simulink model "hex_simulation_standing"  (R2026a)
settings: Solver=VariableStepAuto  StopTime=9
model workspace: external: MATLAB File simscape_data.m (data not in the file)
undefined symbols (not defined in the file or in its folder): smiData, X, Y, Z
libraries: sm_lib x398, nesl_utility x23
(part 7 of 7)

== system hex_simulation_standing/Right Back/Complete_servo_assembly_3_RIGID/Servo_Horn_1_RIGID ==
  ReferenceFrame : sm_lib/Frames and Transforms/Reference Frame
  Solid : sm_lib/Body Elements/File Solid  ExtGeomFileName=servo-horn.step  UnitType=FromFile  ExtGeomFileUnits=m  StepReaderType=HEX  ExportConvexHullGeometry=off  InertiaType=Custom  BasedOnType=DensityFromFile  Density=1000  DensityUnits=kg/m^3  Mass=smiData.Solid(3).mass  MassUnits=kg  CenterOfMass=smiData.Solid(3).CoM  CenterOfMassUnits=mm  MomentsOfInertia=smiData.Solid(3).MoI  MomentsOfInertiaUnits=kg*mm^2  ProductsOfInertia=smiData.Solid(3).PoI  ProductsOfInertiaUnits=kg*mm^2  GraphicType=FromGeometry  MarkerShape=Sphere  MarkerSize=10  GraphicVisPropType=SimpleVisualProperties  GraphicDiffuseColor=smiData.Solid(3).color  GraphicOpacity=smiData.Solid(3).opacity  GraphicSpecularColor=[0.5 0.5 0.5 1.0]  GraphicAmbientColor=[0.15 0.15 0.15 1.0]  GraphicEmissiveColor=[0.0 0.0 0.0 1.0]  GraphicShininess=75  DoExposeReferenceFrame=on  SerializedFrames=<Frames/>
  F : PMIOPort  Side=Left
  connections:
  Solid/RConn1 -- ReferenceFrame/RConn1 -- F/RConn1

== system hex_simulation_standing/Right Front/Complete_servo_assembly_1_RIGID/Assem3Complete_servo_assembly_1_RIGID ==
  ReferenceFrame : sm_lib/Frames and Transforms/Reference Frame
  Transform : sm_lib/Frames and Transforms/Rigid Transform  RotationMethod=ArbitraryAxis  FollAlignAxisA=+X  BaseAlignAxisA=+Y  FollAlignAxisB=+Y  BaseAlignAxisB=+Z  RotationStandardAxis=+Z  RotationAngle=smiData.RigidTransform(74).angle  RotationAngleUnits=rad  RotationArbitraryAxis=smiData.RigidTransform(74).axis  RotationSequenceAxes=FollowerAxes  RotationSequence=XYX  RotationSequenceAngles=[0 0 0]  RotationSequenceAnglesUnits=deg  RotationMatrix=[1 0 0;0 1 0;0 0 1]  Quaternion=[1 0 0 0]  TranslationMethod=Cartesian  TranslationCartesianOffset=smiData.RigidTransform(74).translation  TranslationCartesianOffsetUnits=mm  TranslationStandardAxis=+Z  TranslationStandardOffset=0  TranslationStandardOffsetUnits=m  TranslationROffset=0  TranslationROffsetUnits=m  TranslationThetaOffset=0  TranslationThetaOffsetUnits=deg  TranslationZOffset=0  TranslationZOffsetUnits=m
  F : PMIOPort  Side=Right
  connections:
  ReferenceFrame/RConn1 -- Transform/RConn1
  Transform/LConn1 -- F/RConn1

== system hex_simulation_standing/Right Front/Complete_servo_assembly_1_RIGID/MG996R_servo_1_RIGID ==
  ReferenceFrame : sm_lib/Frames and Transforms/Reference Frame
  Solid : sm_lib/Body Elements/File Solid  ExtGeomFileName=mg996r-servo.step  UnitType=FromFile  ExtGeomFileUnits=m  StepReaderType=HEX  ExportConvexHullGeometry=off  InertiaType=Custom  BasedOnType=DensityFromFile  Density=1000  DensityUnits=kg/m^3  Mass=smiData.Solid(1).mass  MassUnits=kg  CenterOfMass=smiData.Solid(1).CoM  CenterOfMassUnits=mm  MomentsOfInertia=smiData.Solid(1).MoI  MomentsOfInertiaUnits=kg*mm^2  ProductsOfInertia=smiData.Solid(1).PoI  ProductsOfInertiaUnits=kg*mm^2  GraphicType=FromGeometry  MarkerShape=Sphere  MarkerSize=10  GraphicVisPropType=SimpleVisualProperties  GraphicDiffuseColor=smiData.Solid(1).color  GraphicOpacity=smiData.Solid(1).opacity  GraphicSpecularColor=[0.5 0.5 0.5 1.0]  GraphicAmbientColor=[0.15 0.15 0.15 1.0]  GraphicEmissiveColor=[0.0 0.0 0.0 1.0]  GraphicShininess=75  DoExposeReferenceFrame=on  SerializedFrames=<Frames/>
  F : PMIOPort  Side=Left
  connections:
  Solid/RConn1 -- ReferenceFrame/RConn1 -- F/RConn1

== system hex_simulation_standing/Right Front/Complete_servo_assembly_1_RIGID/Opposite_support_for_servo_1_RIGID ==
  ReferenceFrame : sm_lib/Frames and Transforms/Reference Frame
  Solid : sm_lib/Body Elements/File Solid  ExtGeomFileName=opposite-support-for-servo.step  UnitType=FromFile  ExtGeomFileUnits=m  StepReaderType=HEX  ExportConvexHullGeometry=off  InertiaType=Custom  BasedOnType=DensityFromFile  Density=1000  DensityUnits=kg/m^3  Mass=smiData.Solid(2).mass  MassUnits=kg  CenterOfMass=smiData.Solid(2).CoM  CenterOfMassUnits=mm  MomentsOfInertia=smiData.Solid(2).MoI  MomentsOfInertiaUnits=kg*mm^2  ProductsOfInertia=smiData.Solid(2).PoI  ProductsOfInertiaUnits=kg*mm^2  GraphicType=FromGeometry  MarkerShape=Sphere  MarkerSize=10  GraphicVisPropType=SimpleVisualProperties  GraphicDiffuseColor=smiData.Solid(2).color  GraphicOpacity=smiData.Solid(2).opacity  GraphicSpecularColor=[0.5 0.5 0.5 1.0]  GraphicAmbientColor=[0.15 0.15 0.15 1.0]  GraphicEmissiveColor=[0.0 0.0 0.0 1.0]  GraphicShininess=75  DoExposeReferenceFrame=on  SerializedFrames=<Frames/>
  F : PMIOPort  Side=Left
  connections:
  Solid/RConn1 -- ReferenceFrame/RConn1 -- F/RConn1

== system hex_simulation_standing/Right Front/Complete_servo_assembly_1_RIGID/Servo_Horn_1_RIGID ==
  ReferenceFrame : sm_lib/Frames and Transforms/Reference Frame
  Solid : sm_lib/Body Elements/File Solid  ExtGeomFileName=servo-horn.step  UnitType=FromFile  ExtGeomFileUnits=m  StepReaderType=HEX  ExportConvexHullGeometry=off  InertiaType=Custom  BasedOnType=DensityFromFile  Density=1000  DensityUnits=kg/m^3  Mass=smiData.Solid(3).mass  MassUnits=kg  CenterOfMass=smiData.Solid(3).CoM  CenterOfMassUnits=mm  MomentsOfInertia=smiData.Solid(3).MoI  MomentsOfInertiaUnits=kg*mm^2  ProductsOfInertia=smiData.Solid(3).PoI  ProductsOfInertiaUnits=kg*mm^2  GraphicType=FromGeometry  MarkerShape=Sphere  MarkerSize=10  GraphicVisPropType=SimpleVisualProperties  GraphicDiffuseColor=smiData.Solid(3).color  GraphicOpacity=smiData.Solid(3).opacity  GraphicSpecularColor=[0.5 0.5 0.5 1.0]  GraphicAmbientColor=[0.15 0.15 0.15 1.0]  GraphicEmissiveColor=[0.0 0.0 0.0 1.0]  GraphicShininess=75  DoExposeReferenceFrame=on  SerializedFrames=<Frames/>
  F : PMIOPort  Side=Left
  connections:
  Solid/RConn1 -- ReferenceFrame/RConn1 -- F/RConn1

== system hex_simulation_standing/Right Front/Complete_servo_assembly_2_RIGID/Assem3Complete_servo_assembly_1_RIGID ==
  ReferenceFrame : sm_lib/Frames and Transforms/Reference Frame
  Transform : sm_lib/Frames and Transforms/Rigid Transform  RotationMethod=ArbitraryAxis  FollAlignAxisA=+X  BaseAlignAxisA=+Y  FollAlignAxisB=+Y  BaseAlignAxisB=+Z  RotationStandardAxis=+Z  RotationAngle=smiData.RigidTransform(82).angle  RotationAngleUnits=rad  RotationArbitraryAxis=smiData.RigidTransform(82).axis  RotationSequenceAxes=FollowerAxes  RotationSequence=XYX  RotationSequenceAngles=[0 0 0]  RotationSequenceAnglesUnits=deg  RotationMatrix=[1 0 0;0 1 0;0 0 1]  Quaternion=[1 0 0 0]  TranslationMethod=Cartesian  TranslationCartesianOffset=smiData.RigidTransform(82).translation  TranslationCartesianOffsetUnits=mm  TranslationStandardAxis=+Z  TranslationStandardOffset=0  TranslationStandardOffsetUnits=m  TranslationROffset=0  TranslationROffsetUnits=m  TranslationThetaOffset=0  TranslationThetaOffsetUnits=deg  TranslationZOffset=0  TranslationZOffsetUnits=m
  F : PMIOPort  Side=Right
  connections:
  ReferenceFrame/RConn1 -- Transform/RConn1
  Transform/LConn1 -- F/RConn1

== system hex_simulation_standing/Right Front/Complete_servo_assembly_2_RIGID/MG996R_servo_1_RIGID ==
  ReferenceFrame : sm_lib/Frames and Transforms/Reference Frame
  Solid : sm_lib/Body Elements/File Solid  ExtGeomFileName=mg996r-servo.step  UnitType=FromFile  ExtGeomFileUnits=m  StepReaderType=HEX  ExportConvexHullGeometry=off  InertiaType=Custom  BasedOnType=DensityFromFile  Density=1000  DensityUnits=kg/m^3  Mass=smiData.Solid(1).mass  MassUnits=kg  CenterOfMass=smiData.Solid(1).CoM  CenterOfMassUnits=mm  MomentsOfInertia=smiData.Solid(1).MoI  MomentsOfInertiaUnits=kg*mm^2  ProductsOfInertia=smiData.Solid(1).PoI  ProductsOfInertiaUnits=kg*mm^2  GraphicType=FromGeometry  MarkerShape=Sphere  MarkerSize=10  GraphicVisPropType=SimpleVisualProperties  GraphicDiffuseColor=smiData.Solid(1).color  GraphicOpacity=smiData.Solid(1).opacity  GraphicSpecularColor=[0.5 0.5 0.5 1.0]  GraphicAmbientColor=[0.15 0.15 0.15 1.0]  GraphicEmissiveColor=[0.0 0.0 0.0 1.0]  GraphicShininess=75  DoExposeReferenceFrame=on  SerializedFrames=<Frames/>
  F : PMIOPort  Side=Left
  connections:
  Solid/RConn1 -- ReferenceFrame/RConn1 -- F/RConn1

== system hex_simulation_standing/Right Front/Complete_servo_assembly_2_RIGID/Opposite_support_for_servo_1_RIGID ==
  ReferenceFrame : sm_lib/Frames and Transforms/Reference Frame
  Solid : sm_lib/Body Elements/File Solid  ExtGeomFileName=opposite-support-for-servo.step  UnitType=FromFile  ExtGeomFileUnits=m  StepReaderType=HEX  ExportConvexHullGeometry=off  InertiaType=Custom  BasedOnType=DensityFromFile  Density=1000  DensityUnits=kg/m^3  Mass=smiData.Solid(2).mass  MassUnits=kg  CenterOfMass=smiData.Solid(2).CoM  CenterOfMassUnits=mm  MomentsOfInertia=smiData.Solid(2).MoI  MomentsOfInertiaUnits=kg*mm^2  ProductsOfInertia=smiData.Solid(2).PoI  ProductsOfInertiaUnits=kg*mm^2  GraphicType=FromGeometry  MarkerShape=Sphere  MarkerSize=10  GraphicVisPropType=SimpleVisualProperties  GraphicDiffuseColor=smiData.Solid(2).color  GraphicOpacity=smiData.Solid(2).opacity  GraphicSpecularColor=[0.5 0.5 0.5 1.0]  GraphicAmbientColor=[0.15 0.15 0.15 1.0]  GraphicEmissiveColor=[0.0 0.0 0.0 1.0]  GraphicShininess=75  DoExposeReferenceFrame=on  SerializedFrames=<Frames/>
  F : PMIOPort  Side=Left
  connections:
  Solid/RConn1 -- ReferenceFrame/RConn1 -- F/RConn1

== system hex_simulation_standing/Right Front/Complete_servo_assembly_2_RIGID/Servo_Horn_1_RIGID ==
  ReferenceFrame : sm_lib/Frames and Transforms/Reference Frame
  Solid : sm_lib/Body Elements/File Solid  ExtGeomFileName=servo-horn.step  UnitType=FromFile  ExtGeomFileUnits=m  StepReaderType=HEX  ExportConvexHullGeometry=off  InertiaType=Custom  BasedOnType=DensityFromFile  Density=1000  DensityUnits=kg/m^3  Mass=smiData.Solid(3).mass  MassUnits=kg  CenterOfMass=smiData.Solid(3).CoM  CenterOfMassUnits=mm  MomentsOfInertia=smiData.Solid(3).MoI  MomentsOfInertiaUnits=kg*mm^2  ProductsOfInertia=smiData.Solid(3).PoI  ProductsOfInertiaUnits=kg*mm^2  GraphicType=FromGeometry  MarkerShape=Sphere  MarkerSize=10  GraphicVisPropType=SimpleVisualProperties  GraphicDiffuseColor=smiData.Solid(3).color  GraphicOpacity=smiData.Solid(3).opacity  GraphicSpecularColor=[0.5 0.5 0.5 1.0]  GraphicAmbientColor=[0.15 0.15 0.15 1.0]  GraphicEmissiveColor=[0.0 0.0 0.0 1.0]  GraphicShininess=75  DoExposeReferenceFrame=on  SerializedFrames=<Frames/>
  F : PMIOPort  Side=Left
  connections:
  Solid/RConn1 -- ReferenceFrame/RConn1 -- F/RConn1

== system hex_simulation_standing/Right Front/Complete_servo_assembly_3_RIGID/Assem3Complete_servo_assembly_1_RIGID ==
  ReferenceFrame : sm_lib/Frames and Transforms/Reference Frame
  Transform : sm_lib/Frames and Transforms/Rigid Transform  RotationMethod=ArbitraryAxis  FollAlignAxisA=+X  BaseAlignAxisA=+Y  FollAlignAxisB=+Y  BaseAlignAxisB=+Z  RotationStandardAxis=+Z  RotationAngle=smiData.RigidTransform(78).angle  RotationAngleUnits=rad  RotationArbitraryAxis=smiData.RigidTransform(78).axis  RotationSequenceAxes=FollowerAxes  RotationSequence=XYX  RotationSequenceAngles=[0 0 0]  RotationSequenceAnglesUnits=deg  RotationMatrix=[1 0 0;0 1 0;0 0 1]  Quaternion=[1 0 0 0]  TranslationMethod=Cartesian  TranslationCartesianOffset=smiData.RigidTransform(78).translation  TranslationCartesianOffsetUnits=mm  TranslationStandardAxis=+Z  TranslationStandardOffset=0  TranslationStandardOffsetUnits=m  TranslationROffset=0  TranslationROffsetUnits=m  TranslationThetaOffset=0  TranslationThetaOffsetUnits=deg  TranslationZOffset=0  TranslationZOffsetUnits=m
  F : PMIOPort  Side=Right
  connections:
  ReferenceFrame/RConn1 -- Transform/RConn1
  Transform/LConn1 -- F/RConn1

== system hex_simulation_standing/Right Front/Complete_servo_assembly_3_RIGID/MG996R_servo_1_RIGID ==
  ReferenceFrame : sm_lib/Frames and Transforms/Reference Frame
  Solid : sm_lib/Body Elements/File Solid  ExtGeomFileName=mg996r-servo.step  UnitType=FromFile  ExtGeomFileUnits=m  StepReaderType=HEX  ExportConvexHullGeometry=off  InertiaType=Custom  BasedOnType=DensityFromFile  Density=1000  DensityUnits=kg/m^3  Mass=smiData.Solid(1).mass  MassUnits=kg  CenterOfMass=smiData.Solid(1).CoM  CenterOfMassUnits=mm  MomentsOfInertia=smiData.Solid(1).MoI  MomentsOfInertiaUnits=kg*mm^2  ProductsOfInertia=smiData.Solid(1).PoI  ProductsOfInertiaUnits=kg*mm^2  GraphicType=FromGeometry  MarkerShape=Sphere  MarkerSize=10  GraphicVisPropType=SimpleVisualProperties  GraphicDiffuseColor=smiData.Solid(1).color  GraphicOpacity=smiData.Solid(1).opacity  GraphicSpecularColor=[0.5 0.5 0.5 1.0]  GraphicAmbientColor=[0.15 0.15 0.15 1.0]  GraphicEmissiveColor=[0.0 0.0 0.0 1.0]  GraphicShininess=75  DoExposeReferenceFrame=on  SerializedFrames=<Frames/>
  F : PMIOPort  Side=Left
  connections:
  Solid/RConn1 -- ReferenceFrame/RConn1 -- F/RConn1

== system hex_simulation_standing/Right Front/Complete_servo_assembly_3_RIGID/Opposite_support_for_servo_1_RIGID ==
  ReferenceFrame : sm_lib/Frames and Transforms/Reference Frame
  Solid : sm_lib/Body Elements/File Solid  ExtGeomFileName=opposite-support-for-servo.step  UnitType=FromFile  ExtGeomFileUnits=m  StepReaderType=HEX  ExportConvexHullGeometry=off  InertiaType=Custom  BasedOnType=DensityFromFile  Density=1000  DensityUnits=kg/m^3  Mass=smiData.Solid(2).mass  MassUnits=kg  CenterOfMass=smiData.Solid(2).CoM  CenterOfMassUnits=mm  MomentsOfInertia=smiData.Solid(2).MoI  MomentsOfInertiaUnits=kg*mm^2  ProductsOfInertia=smiData.Solid(2).PoI  ProductsOfInertiaUnits=kg*mm^2  GraphicType=FromGeometry  MarkerShape=Sphere  MarkerSize=10  GraphicVisPropType=SimpleVisualProperties  GraphicDiffuseColor=smiData.Solid(2).color  GraphicOpacity=smiData.Solid(2).opacity  GraphicSpecularColor=[0.5 0.5 0.5 1.0]  GraphicAmbientColor=[0.15 0.15 0.15 1.0]  GraphicEmissiveColor=[0.0 0.0 0.0 1.0]  GraphicShininess=75  DoExposeReferenceFrame=on  SerializedFrames=<Frames/>
  F : PMIOPort  Side=Left
  connections:
  Solid/RConn1 -- ReferenceFrame/RConn1 -- F/RConn1

== system hex_simulation_standing/Right Front/Complete_servo_assembly_3_RIGID/Servo_Horn_1_RIGID ==
  ReferenceFrame : sm_lib/Frames and Transforms/Reference Frame
  Solid : sm_lib/Body Elements/File Solid  ExtGeomFileName=servo-horn.step  UnitType=FromFile  ExtGeomFileUnits=m  StepReaderType=HEX  ExportConvexHullGeometry=off  InertiaType=Custom  BasedOnType=DensityFromFile  Density=1000  DensityUnits=kg/m^3  Mass=smiData.Solid(3).mass  MassUnits=kg  CenterOfMass=smiData.Solid(3).CoM  CenterOfMassUnits=mm  MomentsOfInertia=smiData.Solid(3).MoI  MomentsOfInertiaUnits=kg*mm^2  ProductsOfInertia=smiData.Solid(3).PoI  ProductsOfInertiaUnits=kg*mm^2  GraphicType=FromGeometry  MarkerShape=Sphere  MarkerSize=10  GraphicVisPropType=SimpleVisualProperties  GraphicDiffuseColor=smiData.Solid(3).color  GraphicOpacity=smiData.Solid(3).opacity  GraphicSpecularColor=[0.5 0.5 0.5 1.0]  GraphicAmbientColor=[0.15 0.15 0.15 1.0]  GraphicEmissiveColor=[0.0 0.0 0.0 1.0]  GraphicShininess=75  DoExposeReferenceFrame=on  SerializedFrames=<Frames/>
  F : PMIOPort  Side=Left
  connections:
  Solid/RConn1 -- ReferenceFrame/RConn1 -- F/RConn1

== system hex_simulation_standing/Right Middle/Complete_servo_assembly_1_RIGID/Assem3Complete_servo_assembly_1_RIGID ==
  ReferenceFrame : sm_lib/Frames and Transforms/Reference Frame
  Transform : sm_lib/Frames and Transforms/Rigid Transform  RotationMethod=ArbitraryAxis  FollAlignAxisA=+X  BaseAlignAxisA=+Y  FollAlignAxisB=+Y  BaseAlignAxisB=+Z  RotationStandardAxis=+Z  RotationAngle=smiData.RigidTransform(38).angle  RotationAngleUnits=rad  RotationArbitraryAxis=smiData.RigidTransform(38).axis  RotationSequenceAxes=FollowerAxes  RotationSequence=XYX  RotationSequenceAngles=[0 0 0]  RotationSequenceAnglesUnits=deg  RotationMatrix=[1 0 0;0 1 0;0 0 1]  Quaternion=[1 0 0 0]  TranslationMethod=Cartesian  TranslationCartesianOffset=smiData.RigidTransform(38).translation  TranslationCartesianOffsetUnits=mm  TranslationStandardAxis=+Z  TranslationStandardOffset=0  TranslationStandardOffsetUnits=m  TranslationROffset=0  TranslationROffsetUnits=m  TranslationThetaOffset=0  TranslationThetaOffsetUnits=deg  TranslationZOffset=0  TranslationZOffsetUnits=m
  F : PMIOPort  Side=Right
  connections:
  ReferenceFrame/RConn1 -- Transform/RConn1
  Transform/LConn1 -- F/RConn1

== system hex_simulation_standing/Right Middle/Complete_servo_assembly_1_RIGID/MG996R_servo_1_RIGID ==
  ReferenceFrame : sm_lib/Frames and Transforms/Reference Frame
  Solid : sm_lib/Body Elements/File Solid  ExtGeomFileName=mg996r-servo.step  UnitType=FromFile  ExtGeomFileUnits=m  StepReaderType=HEX  ExportConvexHullGeometry=off  InertiaType=Custom  BasedOnType=DensityFromFile  Density=1000  DensityUnits=kg/m^3  Mass=smiData.Solid(1).mass  MassUnits=kg  CenterOfMass=smiData.Solid(1).CoM  CenterOfMassUnits=mm  MomentsOfInertia=smiData.Solid(1).MoI  MomentsOfInertiaUnits=kg*mm^2  ProductsOfInertia=smiData.Solid(1).PoI  ProductsOfInertiaUnits=kg*mm^2  GraphicType=FromGeometry  MarkerShape=Sphere  MarkerSize=10  GraphicVisPropType=SimpleVisualProperties  GraphicDiffuseColor=smiData.Solid(1).color  GraphicOpacity=smiData.Solid(1).opacity  GraphicSpecularColor=[0.5 0.5 0.5 1.0]  GraphicAmbientColor=[0.15 0.15 0.15 1.0]  GraphicEmissiveColor=[0.0 0.0 0.0 1.0]  GraphicShininess=75  DoExposeReferenceFrame=on  SerializedFrames=<Frames/>
  F : PMIOPort  Side=Left
  connections:
  Solid/RConn1 -- ReferenceFrame/RConn1 -- F/RConn1

== system hex_simulation_standing/Right Middle/Complete_servo_assembly_1_RIGID/Opposite_support_for_servo_1_RIGID ==
  ReferenceFrame : sm_lib/Frames and Transforms/Reference Frame
  Solid : sm_lib/Body Elements/File Solid  ExtGeomFileName=opposite-support-for-servo.step  UnitType=FromFile  ExtGeomFileUnits=m  StepReaderType=HEX  ExportConvexHullGeometry=off  InertiaType=Custom  BasedOnType=DensityFromFile  Density=1000  DensityUnits=kg/m^3  Mass=smiData.Solid(2).mass  MassUnits=kg  CenterOfMass=smiData.Solid(2).CoM  CenterOfMassUnits=mm  MomentsOfInertia=smiData.Solid(2).MoI  MomentsOfInertiaUnits=kg*mm^2  ProductsOfInertia=smiData.Solid(2).PoI  ProductsOfInertiaUnits=kg*mm^2  GraphicType=FromGeometry  MarkerShape=Sphere  MarkerSize=10  GraphicVisPropType=SimpleVisualProperties  GraphicDiffuseColor=smiData.Solid(2).color  GraphicOpacity=smiData.Solid(2).opacity  GraphicSpecularColor=[0.5 0.5 0.5 1.0]  GraphicAmbientColor=[0.15 0.15 0.15 1.0]  GraphicEmissiveColor=[0.0 0.0 0.0 1.0]  GraphicShininess=75  DoExposeReferenceFrame=on  SerializedFrames=<Frames/>
  F : PMIOPort  Side=Left
  connections:
  Solid/RConn1 -- ReferenceFrame/RConn1 -- F/RConn1

== system hex_simulation_standing/Right Middle/Complete_servo_assembly_1_RIGID/Servo_Horn_1_RIGID ==
  ReferenceFrame : sm_lib/Frames and Transforms/Reference Frame
  Solid : sm_lib/Body Elements/File Solid  ExtGeomFileName=servo-horn.step  UnitType=FromFile  ExtGeomFileUnits=m  StepReaderType=HEX  ExportConvexHullGeometry=off  InertiaType=Custom  BasedOnType=DensityFromFile  Density=1000  DensityUnits=kg/m^3  Mass=smiData.Solid(3).mass  MassUnits=kg  CenterOfMass=smiData.Solid(3).CoM  CenterOfMassUnits=mm  MomentsOfInertia=smiData.Solid(3).MoI  MomentsOfInertiaUnits=kg*mm^2  ProductsOfInertia=smiData.Solid(3).PoI  ProductsOfInertiaUnits=kg*mm^2  GraphicType=FromGeometry  MarkerShape=Sphere  MarkerSize=10  GraphicVisPropType=SimpleVisualProperties  GraphicDiffuseColor=smiData.Solid(3).color  GraphicOpacity=smiData.Solid(3).opacity  GraphicSpecularColor=[0.5 0.5 0.5 1.0]  GraphicAmbientColor=[0.15 0.15 0.15 1.0]  GraphicEmissiveColor=[0.0 0.0 0.0 1.0]  GraphicShininess=75  DoExposeReferenceFrame=on  SerializedFrames=<Frames/>
  F : PMIOPort  Side=Left
  connections:
  Solid/RConn1 -- ReferenceFrame/RConn1 -- F/RConn1

== system hex_simulation_standing/Right Middle/Complete_servo_assembly_2_RIGID/Assem3Complete_servo_assembly_1_RIGID ==
  ReferenceFrame : sm_lib/Frames and Transforms/Reference Frame
  Transform : sm_lib/Frames and Transforms/Rigid Transform  RotationMethod=ArbitraryAxis  FollAlignAxisA=+X  BaseAlignAxisA=+Y  FollAlignAxisB=+Y  BaseAlignAxisB=+Z  RotationStandardAxis=+Z  RotationAngle=smiData.RigidTransform(42).angle  RotationAngleUnits=rad  RotationArbitraryAxis=smiData.RigidTransform(42).axis  RotationSequenceAxes=FollowerAxes  RotationSequence=XYX  RotationSequenceAngles=[0 0 0]  RotationSequenceAnglesUnits=deg  RotationMatrix=[1 0 0;0 1 0;0 0 1]  Quaternion=[1 0 0 0]  TranslationMethod=Cartesian  TranslationCartesianOffset=smiData.RigidTransform(42).translation  TranslationCartesianOffsetUnits=mm  TranslationStandardAxis=+Z  TranslationStandardOffset=0  TranslationStandardOffsetUnits=m  TranslationROffset=0  TranslationROffsetUnits=m  TranslationThetaOffset=0  TranslationThetaOffsetUnits=deg  TranslationZOffset=0  TranslationZOffsetUnits=m
  F : PMIOPort  Side=Right
  connections:
  ReferenceFrame/RConn1 -- Transform/RConn1
  Transform/LConn1 -- F/RConn1

== system hex_simulation_standing/Right Middle/Complete_servo_assembly_2_RIGID/MG996R_servo_1_RIGID ==
  ReferenceFrame : sm_lib/Frames and Transforms/Reference Frame
  Solid : sm_lib/Body Elements/File Solid  ExtGeomFileName=mg996r-servo.step  UnitType=FromFile  ExtGeomFileUnits=m  StepReaderType=HEX  ExportConvexHullGeometry=off  InertiaType=Custom  BasedOnType=DensityFromFile  Density=1000  DensityUnits=kg/m^3  Mass=smiData.Solid(1).mass  MassUnits=kg  CenterOfMass=smiData.Solid(1).CoM  CenterOfMassUnits=mm  MomentsOfInertia=smiData.Solid(1).MoI  MomentsOfInertiaUnits=kg*mm^2  ProductsOfInertia=smiData.Solid(1).PoI  ProductsOfInertiaUnits=kg*mm^2  GraphicType=FromGeometry  MarkerShape=Sphere  MarkerSize=10  GraphicVisPropType=SimpleVisualProperties  GraphicDiffuseColor=smiData.Solid(1).color  GraphicOpacity=smiData.Solid(1).opacity  GraphicSpecularColor=[0.5 0.5 0.5 1.0]  GraphicAmbientColor=[0.15 0.15 0.15 1.0]  GraphicEmissiveColor=[0.0 0.0 0.0 1.0]  GraphicShininess=75  DoExposeReferenceFrame=on  SerializedFrames=<Frames/>
  F : PMIOPort  Side=Left
  connections:
  Solid/RConn1 -- ReferenceFrame/RConn1 -- F/RConn1

== system hex_simulation_standing/Right Middle/Complete_servo_assembly_2_RIGID/Opposite_support_for_servo_1_RIGID ==
  ReferenceFrame : sm_lib/Frames and Transforms/Reference Frame
  Solid : sm_lib/Body Elements/File Solid  ExtGeomFileName=opposite-support-for-servo.step  UnitType=FromFile  ExtGeomFileUnits=m  StepReaderType=HEX  ExportConvexHullGeometry=off  InertiaType=Custom  BasedOnType=DensityFromFile  Density=1000  DensityUnits=kg/m^3  Mass=smiData.Solid(2).mass  MassUnits=kg  CenterOfMass=smiData.Solid(2).CoM  CenterOfMassUnits=mm  MomentsOfInertia=smiData.Solid(2).MoI  MomentsOfInertiaUnits=kg*mm^2  ProductsOfInertia=smiData.Solid(2).PoI  ProductsOfInertiaUnits=kg*mm^2  GraphicType=FromGeometry  MarkerShape=Sphere  MarkerSize=10  GraphicVisPropType=SimpleVisualProperties  GraphicDiffuseColor=smiData.Solid(2).color  GraphicOpacity=smiData.Solid(2).opacity  GraphicSpecularColor=[0.5 0.5 0.5 1.0]  GraphicAmbientColor=[0.15 0.15 0.15 1.0]  GraphicEmissiveColor=[0.0 0.0 0.0 1.0]  GraphicShininess=75  DoExposeReferenceFrame=on  SerializedFrames=<Frames/>
  F : PMIOPort  Side=Left
  connections:
  Solid/RConn1 -- ReferenceFrame/RConn1 -- F/RConn1

== system hex_simulation_standing/Right Middle/Complete_servo_assembly_2_RIGID/Servo_Horn_1_RIGID ==
  ReferenceFrame : sm_lib/Frames and Transforms/Reference Frame
  Solid : sm_lib/Body Elements/File Solid  ExtGeomFileName=servo-horn.step  UnitType=FromFile  ExtGeomFileUnits=m  StepReaderType=HEX  ExportConvexHullGeometry=off  InertiaType=Custom  BasedOnType=DensityFromFile  Density=1000  DensityUnits=kg/m^3  Mass=smiData.Solid(3).mass  MassUnits=kg  CenterOfMass=smiData.Solid(3).CoM  CenterOfMassUnits=mm  MomentsOfInertia=smiData.Solid(3).MoI  MomentsOfInertiaUnits=kg*mm^2  ProductsOfInertia=smiData.Solid(3).PoI  ProductsOfInertiaUnits=kg*mm^2  GraphicType=FromGeometry  MarkerShape=Sphere  MarkerSize=10  GraphicVisPropType=SimpleVisualProperties  GraphicDiffuseColor=smiData.Solid(3).color  GraphicOpacity=smiData.Solid(3).opacity  GraphicSpecularColor=[0.5 0.5 0.5 1.0]  GraphicAmbientColor=[0.15 0.15 0.15 1.0]  GraphicEmissiveColor=[0.0 0.0 0.0 1.0]  GraphicShininess=75  DoExposeReferenceFrame=on  SerializedFrames=<Frames/>
  F : PMIOPort  Side=Left
  connections:
  Solid/RConn1 -- ReferenceFrame/RConn1 -- F/RConn1

== system hex_simulation_standing/Right Middle/Complete_servo_assembly_3_RIGID/Assem3Complete_servo_assembly_1_RIGID ==
  ReferenceFrame : sm_lib/Frames and Transforms/Reference Frame
  Transform : sm_lib/Frames and Transforms/Rigid Transform  RotationMethod=ArbitraryAxis  FollAlignAxisA=+X  BaseAlignAxisA=+Y  FollAlignAxisB=+Y  BaseAlignAxisB=+Z  RotationStandardAxis=+Z  RotationAngle=smiData.RigidTransform(46).angle  RotationAngleUnits=rad  RotationArbitraryAxis=smiData.RigidTransform(46).axis  RotationSequenceAxes=FollowerAxes  RotationSequence=XYX  RotationSequenceAngles=[0 0 0]  RotationSequenceAnglesUnits=deg  RotationMatrix=[1 0 0;0 1 0;0 0 1]  Quaternion=[1 0 0 0]  TranslationMethod=Cartesian  TranslationCartesianOffset=smiData.RigidTransform(46).translation  TranslationCartesianOffsetUnits=mm  TranslationStandardAxis=+Z  TranslationStandardOffset=0  TranslationStandardOffsetUnits=m  TranslationROffset=0  TranslationROffsetUnits=m  TranslationThetaOffset=0  TranslationThetaOffsetUnits=deg  TranslationZOffset=0  TranslationZOffsetUnits=m
  F : PMIOPort  Side=Right
  connections:
  ReferenceFrame/RConn1 -- Transform/RConn1
  Transform/LConn1 -- F/RConn1

== system hex_simulation_standing/Right Middle/Complete_servo_assembly_3_RIGID/MG996R_servo_1_RIGID ==
  ReferenceFrame : sm_lib/Frames and Transforms/Reference Frame
  Solid : sm_lib/Body Elements/File Solid  ExtGeomFileName=mg996r-servo.step  UnitType=FromFile  ExtGeomFileUnits=m  StepReaderType=HEX  ExportConvexHullGeometry=off  InertiaType=Custom  BasedOnType=DensityFromFile  Density=1000  DensityUnits=kg/m^3  Mass=smiData.Solid(1).mass  MassUnits=kg  CenterOfMass=smiData.Solid(1).CoM  CenterOfMassUnits=mm  MomentsOfInertia=smiData.Solid(1).MoI  MomentsOfInertiaUnits=kg*mm^2  ProductsOfInertia=smiData.Solid(1).PoI  ProductsOfInertiaUnits=kg*mm^2  GraphicType=FromGeometry  MarkerShape=Sphere  MarkerSize=10  GraphicVisPropType=SimpleVisualProperties  GraphicDiffuseColor=smiData.Solid(1).color  GraphicOpacity=smiData.Solid(1).opacity  GraphicSpecularColor=[0.5 0.5 0.5 1.0]  GraphicAmbientColor=[0.15 0.15 0.15 1.0]  GraphicEmissiveColor=[0.0 0.0 0.0 1.0]  GraphicShininess=75  DoExposeReferenceFrame=on  SerializedFrames=<Frames/>
  F : PMIOPort  Side=Left
  connections:
  Solid/RConn1 -- ReferenceFrame/RConn1 -- F/RConn1

== system hex_simulation_standing/Right Middle/Complete_servo_assembly_3_RIGID/Opposite_support_for_servo_1_RIGID ==
  ReferenceFrame : sm_lib/Frames and Transforms/Reference Frame
  Solid : sm_lib/Body Elements/File Solid  ExtGeomFileName=opposite-support-for-servo.step  UnitType=FromFile  ExtGeomFileUnits=m  StepReaderType=HEX  ExportConvexHullGeometry=off  InertiaType=Custom  BasedOnType=DensityFromFile  Density=1000  DensityUnits=kg/m^3  Mass=smiData.Solid(2).mass  MassUnits=kg  CenterOfMass=smiData.Solid(2).CoM  CenterOfMassUnits=mm  MomentsOfInertia=smiData.Solid(2).MoI  MomentsOfInertiaUnits=kg*mm^2  ProductsOfInertia=smiData.Solid(2).PoI  ProductsOfInertiaUnits=kg*mm^2  GraphicType=FromGeometry  MarkerShape=Sphere  MarkerSize=10  GraphicVisPropType=SimpleVisualProperties  GraphicDiffuseColor=smiData.Solid(2).color  GraphicOpacity=smiData.Solid(2).opacity  GraphicSpecularColor=[0.5 0.5 0.5 1.0]  GraphicAmbientColor=[0.15 0.15 0.15 1.0]  GraphicEmissiveColor=[0.0 0.0 0.0 1.0]  GraphicShininess=75  DoExposeReferenceFrame=on  SerializedFrames=<Frames/>
  F : PMIOPort  Side=Left
  connections:
  Solid/RConn1 -- ReferenceFrame/RConn1 -- F/RConn1

== system hex_simulation_standing/Right Middle/Complete_servo_assembly_3_RIGID/Servo_Horn_1_RIGID ==
  ReferenceFrame : sm_lib/Frames and Transforms/Reference Frame
  Solid : sm_lib/Body Elements/File Solid  ExtGeomFileName=servo-horn.step  UnitType=FromFile  ExtGeomFileUnits=m  StepReaderType=HEX  ExportConvexHullGeometry=off  InertiaType=Custom  BasedOnType=DensityFromFile  Density=1000  DensityUnits=kg/m^3  Mass=smiData.Solid(3).mass  MassUnits=kg  CenterOfMass=smiData.Solid(3).CoM  CenterOfMassUnits=mm  MomentsOfInertia=smiData.Solid(3).MoI  MomentsOfInertiaUnits=kg*mm^2  ProductsOfInertia=smiData.Solid(3).PoI  ProductsOfInertiaUnits=kg*mm^2  GraphicType=FromGeometry  MarkerShape=Sphere  MarkerSize=10  GraphicVisPropType=SimpleVisualProperties  GraphicDiffuseColor=smiData.Solid(3).color  GraphicOpacity=smiData.Solid(3).opacity  GraphicSpecularColor=[0.5 0.5 0.5 1.0]  GraphicAmbientColor=[0.15 0.15 0.15 1.0]  GraphicEmissiveColor=[0.0 0.0 0.0 1.0]  GraphicShininess=75  DoExposeReferenceFrame=on  SerializedFrames=<Frames/>
  F : PMIOPort  Side=Left
  connections:
  Solid/RConn1 -- ReferenceFrame/RConn1 -- F/RConn1

== matlab function hex_simulation_standing/IK ==
  data: coords input; thetas output
function thetas = fcn(coords)
% Input: [x y z] in millimetres, relative to shoulder horn center.
% Output: absolute Simscape joint commands in radians.
% Order: [shoulder, hip, knee]

% Geometry: initial approximation from CAD measurements
a = 60.00;       % Hip-to-knee length in bending plane
b = 156.33;      % Knee-to-foot length in bending plane
L = 31.80;      % Shoulder-to-hip outward offset
hipZ = -15.15;  % Hip is below shoulder

% Geometric angles in the measured reference pose
phi0   = deg2rad(-0.43);
delta0 = deg2rad(-21.09);

% Simscape commands for that reference pose
qShoulder0 = pi;
qHip0      = 3*pi/2;
qKnee0     = 0;

% Requested foot position
x = coords(1);
y = coords(2);
z = coords(3);

% Shoulder sweep and target relative to hip
psi = atan2(y, x);
d = hypot(x, y) - L;
v = z - hipZ;

% Check this outward-reaching branch
assert(d > 0, 'Target must be outward of the hip.');

% Cosine of the relative knee angle
D = (d*d + v*v - a*a - b*b) / (2*a*b);

% Reject unreachable targets; clamp only numerical roundoff
assert(D >= -1-1e-9 && D <= 1+1e-9, ...
    'Foot target is outside the geometric workspace.');
D = max(-1, min(1, D));

% Choose the knee-bent-down branch
delta = -acos(D);

% Upper-leg elevation above horizontal
phi = atan2(v, d) ...
    - atan2(b*sin(delta), a + b*cos(delta));

% Convert geometric angles to Simscape joint commands
qShoulder = qShoulder0 + psi;
qHip     = qHip0 - (phi - phi0);
qKnee    = qKnee0 + (delta - delta0);

thetas = [qShoulder, qHip, qKnee];
end

== matlab function hex_simulation_standing/Foot Trajectory ==
  data: t input; coords output
function coords = fcn(t)
phaseOffset = 0;  % Fraction of one complete cycle
% Foot coordinates in mm; time in seconds.

x0 = 150;
z0 = -120;

stepLength = 20;
liftHeight = 10;

Tstance = 2;  % Seconds moving backward
Tswing  = 2;  % Seconds returning through the air
startTime = 1;

% Direction of forward travel in this leg's local XY plane.
headingDeg = 50;

center = [x0, 0, z0];
direction = [cosd(headingDeg), sind(headingDeg), 0];

front = center + (stepLength/2)*direction;
rear  = center - (stepLength/2)*direction;

Tcycle = Tstance + Tswing;

% Freeze the gait clock during the initial hold.
tMove = max(0, t - startTime);

% Each group uses the same clock with a different phase.
tau = mod(tMove + phaseOffset*Tcycle, Tcycle);

if tau < Tstance
    % STANCE: straight line from front to rear.
    u = tau/Tstance;
    s = 10*u^3 - 15*u^4 + 6*u^5;

    coords = (1-s)*front + s*rear;

else
    % SWING: curved return from rear to front.
    u = (tau - Tstance)/Tswing;
    s = 10*u^3 - 15*u^4 + 6*u^5;

    P0 = rear;
    P1 = rear  + [0, 0, 4*liftHeight/3];
    P2 = front + [0, 0, 4*liftHeight/3];
    P3 = front;

    coords = (1-s)^3*P0 ...
           + 3*(1-s)^2*s*P1 ...
           + 3*(1-s)*s^2*P2 ...
           + s^3*P3;
end
end

== matlab function hex_simulation_standing/IK1 ==
  data: coords input; thetas output
function thetas = fcn(coords)
% Input: [x y z] in millimetres, relative to shoulder horn center.
% Output: absolute Simscape joint commands in radians.
% Order: [shoulder, hip, knee]

% Geometry: initial approximation from CAD measurements
a = 60.00;       % Hip-to-knee length in bending plane
b = 156.33;      % Knee-to-foot length in bending plane
L = 31.80;      % Shoulder-to-hip outward offset
hipZ = -15.15;  % Hip is below shoulder

% Geometric angles in the measured reference pose
phi0   = deg2rad(-0.43);
delta0 = deg2rad(-21.09);

% Simscape commands for that reference pose
qShoulder0 = pi;
qHip0      = 3*pi/2;
qKnee0     = 0;

% Requested foot position
x = coords(1);
y = coords(2);
z = coords(3);

% Shoulder sweep and target relative to hip
psi = atan2(y, x);
d = hypot(x, y) - L;
v = z - hipZ;

% Check this outward-reaching branch
assert(d > 0, 'Target must be outward of the hip.');

% Cosine of the relative knee angle
D = (d*d + v*v - a*a - b*b) / (2*a*b);

% Reject unreachable targets; clamp only numerical roundoff
assert(D >= -1-1e-9 && D <= 1+1e-9, ...
    'Foot target is outside the geometric workspace.');
D = max(-1, min(1, D));

% Choose the knee-bent-down branch
delta = -acos(D);

% Upper-leg elevation above horizontal
phi = atan2(v, d) ...
    - atan2(b*sin(delta), a + b*cos(delta));

% Convert geometric angles to Simscape joint commands
qShoulder = qShoulder0 + psi;
qHip     = qHip0 - (phi - phi0);
qKnee    = qKnee0 + (delta - delta0);

thetas = [qShoulder, qHip, qKnee];
end

== matlab function hex_simulation_standing/Foot Trajectory1 ==
  data: t input; coords output
function coords = fcn(t)
phaseOffset = 0.5;  % Fraction of one complete cycle
% Foot coordinates in mm; time in seconds.

x0 = 150;
z0 = -120;

stepLength = 20;
liftHeight = 10;

Tstance = 2;  % Seconds moving backward
Tswing  = 2;  % Seconds returning through the air
startTime = 1;

% Direction of forward travel in this leg's local XY plane.
headingDeg = 90;

center = [x0, 0, z0];
direction = [cosd(headingDeg), sind(headingDeg), 0];

front = center + (stepLength/2)*direction;
rear  = center - (stepLength/2)*direction;

Tcycle = Tstance + Tswing;

% Freeze the gait clock during the initial hold.
tMove = max(0, t - startTime);

% Each group uses the same clock with a different phase.
tau = mod(tMove + phaseOffset*Tcycle, Tcycle);

if tau < Tstance
    % STANCE: straight line from front to rear.
    u = tau/Tstance;
    s = 10*u^3 - 15*u^4 + 6*u^5;

    coords = (1-s)*front + s*rear;

else
    % SWING: curved return from rear to front.
    u = (tau - Tstance)/Tswing;
    s = 10*u^3 - 15*u^4 + 6*u^5;

    P0 = rear;
    P1 = rear  + [0, 0, 4*liftHeight/3];
    P2 = front + [0, 0, 4*liftHeight/3];
    P3 = front;

    coords = (1-s)^3*P0 ...
           + 3*(1-s)^2*s*P1 ...
           + 3*(1-s)*s^2*P2 ...
           + s^3*P3;
end
end

== matlab function hex_simulation_standing/IK2 ==
  data: coords input; thetas output
function thetas = fcn(coords)
% Input: [x y z] in millimetres, relative to shoulder horn center.
% Output: absolute Simscape joint commands in radians.
% Order: [shoulder, hip, knee]

% Geometry: initial approximation from CAD measurements
a = 60.00;       % Hip-to-knee length in bending plane
b = 156.33;      % Knee-to-foot length in bending plane
L = 31.80;      % Shoulder-to-hip outward offset
hipZ = -15.15;  % Hip is below shoulder

% Geometric angles in the measured reference pose
phi0   = deg2rad(-0.43);
delta0 = deg2rad(-21.09);

% Simscape commands for that reference pose
qShoulder0 = pi;
qHip0      = 3*pi/2;
qKnee0     = 0;

% Requested foot position
x = coords(1);
y = coords(2);
z = coords(3);

% Shoulder sweep and target relative to hip
psi = atan2(y, x);
d = hypot(x, y) - L;
v = z - hipZ;

% Check this outward-reaching branch
assert(d > 0, 'Target must be outward of the hip.');

% Cosine of the relative knee angle
D = (d*d + v*v - a*a - b*b) / (2*a*b);

% Reject unreachable targets; clamp only numerical roundoff
assert(D >= -1-1e-9 && D <= 1+1e-9, ...
    'Foot target is outside the geometric workspace.');
D = max(-1, min(1, D));

% Choose the knee-bent-down branch
delta = -acos(D);

% Upper-leg elevation above horizontal
phi = atan2(v, d) ...
    - atan2(b*sin(delta), a + b*cos(delta));

% Convert geometric angles to Simscape joint commands
qShoulder = qShoulder0 + psi;
qHip     = qHip0 - (phi - phi0);
qKnee    = qKnee0 + (delta - delta0);

thetas = [qShoulder, qHip, qKnee];
end

== matlab function hex_simulation_standing/IK3 ==
  data: coords input; thetas output
function thetas = fcn(coords)
% Input: [x y z] in millimetres, relative to shoulder horn center.
% Output: absolute Simscape joint commands in radians.
% Order: [shoulder, hip, knee]

% Geometry: initial approximation from CAD measurements
a = 60.00;       % Hip-to-knee length in bending plane
b = 156.33;      % Knee-to-foot length in bending plane
L = 31.80;      % Shoulder-to-hip outward offset
hipZ = -15.15;  % Hip is below shoulder

% Geometric angles in the measured reference pose
phi0   = deg2rad(-0.43);
delta0 = deg2rad(-21.09);

% Simscape commands for that reference pose
qShoulder0 = pi;
qHip0      = 3*pi/2;
qKnee0     = 0;

% Requested foot position
x = coords(1);
y = coords(2);
z = coords(3);

% Shoulder sweep and target relative to hip
psi = atan2(y, x);
d = hypot(x, y) - L;
v = z - hipZ;

% Check this outward-reaching branch
assert(d > 0, 'Target must be outward of the hip.');

% Cosine of the relative knee angle
D = (d*d + v*v - a*a - b*b) / (2*a*b);

% Reject unreachable targets; clamp only numerical roundoff
assert(D >= -1-1e-9 && D <= 1+1e-9, ...
    'Foot target is outside the geometric workspace.');
D = max(-1, min(1, D));

% Choose the knee-bent-down branch
delta = -acos(D);

% Upper-leg elevation above horizontal
phi = atan2(v, d) ...
    - atan2(b*sin(delta), a + b*cos(delta));

% Convert geometric angles to Simscape joint commands
qShoulder = qShoulder0 + psi;
qHip     = qHip0 - (phi - phi0);
qKnee    = qKnee0 + (delta - delta0);

thetas = [qShoulder, qHip, qKnee];
end

== matlab function hex_simulation_standing/IK4 ==
  data: coords input; thetas output
function thetas = fcn(coords)
% Input: [x y z] in millimetres, relative to shoulder horn center.
% Output: absolute Simscape joint commands in radians.
% Order: [shoulder, hip, knee]

% Geometry: initial approximation from CAD measurements
a = 60.00;       % Hip-to-knee length in bending plane
b = 156.33;      % Knee-to-foot length in bending plane
L = 31.80;      % Shoulder-to-hip outward offset
hipZ = -15.15;  % Hip is below shoulder

% Geometric angles in the measured reference pose
phi0   = deg2rad(-0.43);
delta0 = deg2rad(-21.09);

% Simscape commands for that reference pose
qShoulder0 = pi;
qHip0      = 3*pi/2;
qKnee0     = 0;

% Requested foot position
x = coords(1);
y = coords(2);
z = coords(3);

% Shoulder sweep and target relative to hip
psi = atan2(y, x);
d = hypot(x, y) - L;
v = z - hipZ;

% Check this outward-reaching branch
assert(d > 0, 'Target must be outward of the hip.');

% Cosine of the relative knee angle
D = (d*d + v*v - a*a - b*b) / (2*a*b);

% Reject unreachable targets; clamp only numerical roundoff
assert(D >= -1-1e-9 && D <= 1+1e-9, ...
    'Foot target is outside the geometric workspace.');
D = max(-1, min(1, D));

% Choose the knee-bent-down branch
delta = -acos(D);

% Upper-leg elevation above horizontal
phi = atan2(v, d) ...
    - atan2(b*sin(delta), a + b*cos(delta));

% Convert geometric angles to Simscape joint commands
qShoulder = qShoulder0 + psi;
qHip     = qHip0 - (phi - phi0);
qKnee    = qKnee0 + (delta - delta0);

thetas = [qShoulder, qHip, qKnee];
end

== matlab function hex_simulation_standing/IK5 ==
  data: coords input; thetas output
function thetas = fcn(coords)
% Input: [x y z] in millimetres, relative to shoulder horn center.
% Output: absolute Simscape joint commands in radians.
% Order: [shoulder, hip, knee]

% Geometry: initial approximation from CAD measurements
a = 60.00;       % Hip-to-knee length in bending plane
b = 156.33;      % Knee-to-foot length in bending plane
L = 31.80;      % Shoulder-to-hip outward offset
hipZ = -15.15;  % Hip is below shoulder

% Geometric angles in the measured reference pose
phi0   = deg2rad(-0.43);
delta0 = deg2rad(-21.09);

% Simscape commands for that reference pose
qShoulder0 = pi;
qHip0      = 3*pi/2;
qKnee0     = 0;

% Requested foot position
x = coords(1);
y = coords(2);
z = coords(3);

% Shoulder sweep and target relative to hip
psi = atan2(y, x);
d = hypot(x, y) - L;
v = z - hipZ;

% Check this outward-reaching branch
assert(d > 0, 'Target must be outward of the hip.');

% Cosine of the relative knee angle
D = (d*d + v*v - a*a - b*b) / (2*a*b);

% Reject unreachable targets; clamp only numerical roundoff
assert(D >= -1-1e-9 && D <= 1+1e-9, ...
    'Foot target is outside the geometric workspace.');
D = max(-1, min(1, D));

% Choose the knee-bent-down branch
delta = -acos(D);

% Upper-leg elevation above horizontal
phi = atan2(v, d) ...
    - atan2(b*sin(delta), a + b*cos(delta));

% Convert geometric angles to Simscape joint commands
qShoulder = qShoulder0 + psi;
qHip     = qHip0 - (phi - phi0);
qKnee    = qKnee0 + (delta - delta0);

thetas = [qShoulder, qHip, qKnee];
end

== matlab function hex_simulation_standing/Foot Trajectory2 ==
  data: t input; coords output
function coords = fcn(t)
phaseOffset = 0;  % Fraction of one complete cycle
% Foot coordinates in mm; time in seconds.

x0 = 150;
z0 = -120;

stepLength = 20;
liftHeight = 10;

Tstance = 2;  % Seconds moving backward
Tswing  = 2;  % Seconds returning through the air
startTime = 1;

% Direction of forward travel in this leg's local XY plane.
headingDeg = 130;

center = [x0, 0, z0];
direction = [cosd(headingDeg), sind(headingDeg), 0];

front = center + (stepLength/2)*direction;
rear  = center - (stepLength/2)*direction;

Tcycle = Tstance + Tswing;

% Freeze the gait clock during the initial hold.
tMove = max(0, t - startTime);

% Each group uses the same clock with a different phase.
tau = mod(tMove + phaseOffset*Tcycle, Tcycle);

if tau < Tstance
    % STANCE: straight line from front to rear.
    u = tau/Tstance;
    s = 10*u^3 - 15*u^4 + 6*u^5;

    coords = (1-s)*front + s*rear;

else
    % SWING: curved return from rear to front.
    u = (tau - Tstance)/Tswing;
    s = 10*u^3 - 15*u^4 + 6*u^5;

    P0 = rear;
    P1 = rear  + [0, 0, 4*liftHeight/3];
    P2 = front + [0, 0, 4*liftHeight/3];
    P3 = front;

    coords = (1-s)^3*P0 ...
           + 3*(1-s)^2*s*P1 ...
           + 3*(1-s)*s^2*P2 ...
           + s^3*P3;
end
end

== matlab function hex_simulation_standing/Foot Trajectory3 ==
  data: t input; coords output
function coords = fcn(t)
phaseOffset = 0.5;  % Fraction of one complete cycle
% Foot coordinates in mm; time in seconds.

x0 = 150;
z0 = -120;

stepLength = 20;
liftHeight = 10;

Tstance = 2;  % Seconds moving backward
Tswing  = 2;  % Seconds returning through the air
startTime = 1;

% Direction of forward travel in this leg's local XY plane.
headingDeg = -130;

center = [x0, 0, z0];
direction = [cosd(headingDeg), sind(headingDeg), 0];

front = center + (stepLength/2)*direction;
rear  = center - (stepLength/2)*direction;

Tcycle = Tstance + Tswing;

% Freeze the gait clock during the initial hold.
tMove = max(0, t - startTime);

% Each group uses the same clock with a different phase.
tau = mod(tMove + phaseOffset*Tcycle, Tcycle);

if tau < Tstance
    % STANCE: straight line from front to rear.
    u = tau/Tstance;
    s = 10*u^3 - 15*u^4 + 6*u^5;

    coords = (1-s)*front + s*rear;

else
    % SWING: curved return from rear to front.
    u = (tau - Tstance)/Tswing;
    s = 10*u^3 - 15*u^4 + 6*u^5;

    P0 = rear;
    P1 = rear  + [0, 0, 4*liftHeight/3];
    P2 = front + [0, 0, 4*liftHeight/3];
    P3 = front;

    coords = (1-s)^3*P0 ...
           + 3*(1-s)^2*s*P1 ...
           + 3*(1-s)*s^2*P2 ...
           + s^3*P3;
end
end

== matlab function hex_simulation_standing/Foot Trajectory4 ==
  data: t input; coords output
function coords = fcn(t)
phaseOffset = 0;  % Fraction of one complete cycle
% Foot coordinates in mm; time in seconds.

x0 = 150;
z0 = -120;

stepLength = 20;
liftHeight = 10;

Tstance = 2;  % Seconds moving backward
Tswing  = 2;  % Seconds returning through the air
startTime = 1;

% Direction of forward travel in this leg's local XY plane.
headingDeg = -90;

center = [x0, 0, z0];
direction = [cosd(headingDeg), sind(headingDeg), 0];

front = center + (stepLength/2)*direction;
rear  = center - (stepLength/2)*direction;

Tcycle = Tstance + Tswing;

% Freeze the gait clock during the initial hold.
tMove = max(0, t - startTime);

% Each group uses the same clock with a different phase.
tau = mod(tMove + phaseOffset*Tcycle, Tcycle);

if tau < Tstance
    % STANCE: straight line from front to rear.
    u = tau/Tstance;
    s = 10*u^3 - 15*u^4 + 6*u^5;

    coords = (1-s)*front + s*rear;

else
    % SWING: curved return from rear to front.
    u = (tau - Tstance)/Tswing;
    s = 10*u^3 - 15*u^4 + 6*u^5;

    P0 = rear;
    P1 = rear  + [0, 0, 4*liftHeight/3];
    P2 = front + [0, 0, 4*liftHeight/3];
    P3 = front;

    coords = (1-s)^3*P0 ...
           + 3*(1-s)^2*s*P1 ...
           + 3*(1-s)*s^2*P2 ...
           + s^3*P3;
end
end

== matlab function hex_simulation_standing/Foot Trajectory5 ==
  data: t input; coords output
function coords = fcn(t)
phaseOffset = 0.5;  % Fraction of one complete cycle
% Foot coordinates in mm; time in seconds.

x0 = 150;
z0 = -120;

stepLength = 20;
liftHeight = 10;

Tstance = 2;  % Seconds moving backward
Tswing  = 2;  % Seconds returning through the air
startTime = 1;

% Direction of forward travel in this leg's local XY plane.
headingDeg = -50;

center = [x0, 0, z0];
direction = [cosd(headingDeg), sind(headingDeg), 0];

front = center + (stepLength/2)*direction;
rear  = center - (stepLength/2)*direction;

Tcycle = Tstance + Tswing;

% Freeze the gait clock during the initial hold.
tMove = max(0, t - startTime);

% Each group uses the same clock with a different phase.
tau = mod(tMove + phaseOffset*Tcycle, Tcycle);

if tau < Tstance
    % STANCE: straight line from front to rear.
    u = tau/Tstance;
    s = 10*u^3 - 15*u^4 + 6*u^5;

    coords = (1-s)*front + s*rear;

else
    % SWING: curved return from rear to front.
    u = (tau - Tstance)/Tswing;
    s = 10*u^3 - 15*u^4 + 6*u^5;

    P0 = rear;
    P1 = rear  + [0, 0, 4*liftHeight/3];
    P2 = front + [0, 0, 4*liftHeight/3];
    P3 = front;

    coords = (1-s)^3*P0 ...
           + 3*(1-s)^2*s*P1 ...
           + 3*(1-s)*s^2*P2 ...
           + s^3*P3;
end
end

== matlab function hex_simulation_standing/Body Travel ==
  data: t input; distance_mm output
function distance_mm = fcn(t)
% Forward displacement from the body's initial position.

stepLength = 20;   % Must match the foot trajectories
Tstance = 2;      % Must match the foot trajectories
startTime = 1;    % Must match the foot trajectories

tMove = max(0, t - startTime);

% Number of completed stance intervals.
n = floor(tMove / Tstance);

% Progress through the current stance interval: 0 to 1.
u = (tMove - n*Tstance) / Tstance;

% Same smooth timing used by the supporting feet.
s = 10*u^3 - 15*u^4 + 6*u^5;

distance_mm = stepLength * (n + s);
end
